simulink model "Particle_swarm_based_PV_MPPT"  (R2017a)
settings: Solver=ode45  StartTime=0.0  StopTime=1  RelTol=1e-3  EnableMultiTasking=on
undefined symbols (not defined in the file): dEgdT, EgRef, gcbh, k1, Rsh_array5pc, sigbuilder_block, sps_rtmsupport, Tref_K, Ts, VT_ref
libraries: powerlib x16, spsPVarrayModel x3, simulink x1, powerlib_meascontrol x1
(part 2 of 6)

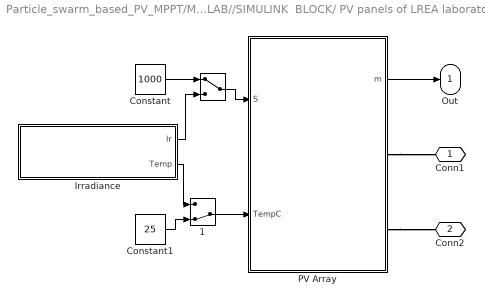
== system Particle_swarm_based_PV_MPPT/MATLAB//SIMULINK  BLOCK/	PV panels of LREA laboratory  ==
  "      " : ManualSwitch
  "      1" : ManualSwitch  CurrentSetting=0
  Constant : Constant  Value=1000
  Constant1 : Constant  Value=25
  "Irradiance " : Subsystem  Tag=STV Subsys  LoadFcn=sigbuilder_block('load');  StartFcn=sigbuilder_block('start');  StopFcn=sigbuilder_block('stop');  ClipboardFcn=sigbuilder_block('clipboard');  mask(Sigbuilder block){tuvar=[0:10]}
      mask help: Sigbuilder GUI
      mask init:
      | if ~strcmp(get_param(bdroot(gcbh),'SimulationStatus'),'stopped') tuvar = sigbuilder_block('maskInit'); end
      settings: CopyFcn=sigbuilder_block('copy');  DeleteFcn=sigbuilder_block('delete');  ModelCloseFcn=sigbuilder_block('modelClose');  PreSaveFcn=sigbuilder_block('preSave');  PauseFcn=sigbuilder_block('pause')  ContinueFcn=sigbuilder_block('continue')  NameChangeFcn=sigbuilder_block('namechange');  OpenFcn=sigbuilder_block('open',[6 30 1188 546.75 ]);  CloseFcn=sigbuilder_block('close');
      mask Display: plot(0, 0, 100, 100,[2, 2, 32, 32, 2], [68, 8, 8, 68, 68],[32, 2], [38, 38], [32, 19, 2],[53, 60, 44], [32, 17, 17, 2],[16, 16, 31, 31]);txt = getActiveGroup(gcbh);text(2, 100, txt,'verticalAlignment', 'top');
  PV Array : Subsystem  AncestorBlock=re_lib/Solar/PV Array  DialogController=POWERSYS.PowerSysDialog  LoadFcn=sps_rtmsupport('LoadFcn',gcbh);  StartFcn=sps_rtmsupport('StartFcn',gcbh);  StopFcn=sps_rtmsupport('StopFcn',gcbh);  mask(PV array){Npar=1, Nser=2, PlotType=array @ 25 deg.C & specified irradiances, S_vec=[1000 800 600 400 ], Temp_C_vec=[ 25 ], ModuleName=User-defined, PlotWhenSelected=off, Pm=200.22, Ncell=60, Voc=57.6, Isc=4.6, Vm=47, Im=4.26, beta_Voc_pc=-0.35502, alpha_Isc_pc=0.06, beta_Voc=-0.20449, alpha_Isc=0.00276, IL=4.6092, I0=1.2872e-10, nI=1.5395, Rsh=412.7019, Rs=0.82756, BAL=on, Tc=1e-6, Tfilter=5e-5}
      mask prompts: Npar "Parallel strings"; Nser "Series-connected modules per string"; S_vec "Irradiances (W/m2)"; Temp_C_vec "T_cell (deg. C)"; ModuleName "Module:"; PlotWhenSelected "Plot I-V and P-V characteristics when a module is selected"; Pm "Maximum Power (W)"; Ncell "Cells per module (Ncell)"; Voc "Open circuit voltage  Voc (V)"; Isc "Short-circuit current Isc (A)"; Vm "Voltage at maximum power point Vmp (V)"; Im "Current at maximum power point Imp (A)"; beta_Voc_pc "Temperature coefficient of Voc (%/deg.C)"; alpha_Isc_pc "Temperature coefficient of Isc (%/deg.C)"; beta_Voc "Temperature coefficient of Voc (V/deg.C)"; alpha_Isc "Temperature coefficient of Isc (A/deg.C)"; IL "Light-generated current IL (A)"; I0 "Diode saturation current I0 (A)"; nI "Diode ideality factor"; Rsh "Shunt resistance Rsh (ohms)"; Rs "Series resistance Rs (ohms)"; BAL "Break algebaic loop in internal model"; Tc "Time constant (s)"; Tfilter "Time constant (s)"
      mask help:
      | Implements a PV array built of strings of PV modules connected in parallel. Each string consists of modules connected in series.
      | Allows modeling of a variety of preset PV modules available from NREL System Advisor Model (Jan. 2014) as well as user-defined PV module.
      |
      | Input 1 = Sun irradiance, in W/m2, and input 2 = Cell temperature, in deg.C.
      mask init:
      | Block = gcb;
      | [k,k1,q,Tref_C,Tref_K,EgRef,dEgdT,Rsh_array5pc,VT_ref,Tsf,Tf,WantBlockChoice] = PVArrayInit(Block, ModuleName, Nser, Npar, Ncell, Rsh, nI, Tfilter);
      | powericon('SetInternalModels','set',Block,WantBlockChoice);
      | sps_rtmsupport('parametereditingmodes',Block, [3 6 7 23]);
      settings: CopyFcn=sps_rtmsupport('CopyFcn',gcbh);  DeleteFcn=sps_rtmsupport('DeleteFcn',gcbh);  UndoDeleteFcn=sps_rtmsupport('UndoDeleteFcn',gcbh);  ModelCloseFcn=sps_rtmsupport('ModelCloseFcn',gcbh);  PreSaveFcn=sps_rtmsupport('PreSaveFcn',gcbh);  PostSaveFcn=sps_rtmsupport('PostSaveFcn',gcbh);  NameChangeFcn=sps_rtmsupport('NameChangeFcn',gcbh);  PreCopyFcn=sps_rtmsupport('PreCopyFcn',gcbh);  CloseFcn=sps_rtmsupport('CloseFcn',gcbh);  PreDeleteFcn=sps_rtmsupport('PreDeleteFcn',gcbh);
      settings: AttributesFormatString=|
      | %<ModuleName>
      | %<Nser>-module string
      | %<Npar> parallel strings
      settings: OpenFcn=|
      | %assignin('base','PVMaskOpening',1);
      | %open_system(gcb,'mask')
      | %assignin('base','PVMaskOpening',0);
      | sps_rtmsupport('OpenFcn',gcbh, [3 6 7 23]);
      mask Help: helpview(psbhelp);
      mask TypeOptions PlotType: one module @ 25 deg.C & specified irradiances | array @ 25 deg.C & specified irradiances | array @ 1000 W/m2 & specified temperatures
      mask Callback PlotType: PVArrayCback(gcb)
